simulink model "YMBOX_Control_Core"  (R2024b)
settings: Solver=FixedStepDiscrete  StartTime=0.0  StopTime=3  RelTol=1e-3
PreLoadFcn:
  | run(fullfile(fileparts(get_param(bdroot,'FileName')), 'YMBOX_Deluxe_init.m'));
InitFcn:
  | YMBOX_InitializeModel('core',bdroot);
model workspace (MAT data in the model file):
  KuMDAS_ObserverBuildVariant : Simulink.Parameter (value not decoded)
undefined symbols (not defined in the file or in its folder): CeMDSM_DrvModeIfStart_enum, CeMDSM_DrvModeSpdSens_enum, CeMDSM_DrvModeSpdSmo_enum, CeMDSM_DrvModeTrq_enum, Cf_CONTROL_TASK_TIME_S, KbMDAS_SmoDeadTimeCompEnable_flg, KbMDSA_ActiveInverterCompEnable_flg, KbMDSA_UnifiedVoltageLimitEnable_flg, KbMDSP_DCBusVoltReportFilterEnable_flg, KbMDTM_DAxisPriorityInFW_flg, KbMDTM_FieldWeakeningEnable_flg, KbMDTM_FinalIqAntiWindupEnable_flg, KbMDTM_SensorlessFieldWeakeningEnable_flg, KbMDTM_TorquePriorityBelowBase_flg, KbMDTM_UnifiedConstraintEnable_flg, KfMDAS_ControlCountToElecRad_NULL, KfMDAS_IfAccel_rpms, KfMDAS_IfAlignTime_s, KfMDAS_IfBlendTime_s, KfMDAS_IfSwitchSpd_rpm, KfMDAS_NativeCountToMechRad_NULL, KfMDAS_ObserverExitRatio_NULL, KfMDAS_SlsCtrlPeriod_s, KfMDAS_SlsEAngleInit_rad, KfMDAS_SlsElecSpdMax_rads, KfMDAS_SlsElecSpdMin_rads, KfMDAS_SlsTwoPi_rad, KfMDAS_SmoAngleOffset_rad, KfMDAS_SmoCurrentZohCoefA_NULL, KfMDAS_SmoCurrentZohCoefB_AperV, KfMDAS_SmoDeadTimeCurrentBoundary_A, KfMDAS_SmoDeadTimeDuty_NULL, KfMDAS_SmoDeadTimePolarity_NULL, KfMDAS_SmoDeviceDrop_V, KfMDAS_SmoEmfLpfCoefA_NULL, KfMDAS_SmoEmfLpfCoefB_NULL, KfMDAS_SmoEmfLpfInvPole_s, KfMDAS_SmoErrBoundaryMax_A, KfMDAS_SmoErrBoundarySpan_A, KfMDAS_SmoGainSchedAlpha_NULL, KfMDAS_SmoGainSchedAngleComp_rad, KfMDAS_SmoGainSchedEmfLow_V, KfMDAS_SmoGainSchedInvSpan_PerV, KfMDAS_SmoLdMinusLq_H, KfMDAS_SmoPllKiTs_NULL, KfMDAS_SmoPllKp_NULL, KfMDAS_SmoPllMinEmf_V, KfMDAS_SmoPllSpeedLpfAlpha_NULL, KfMDAS_SmoSlideGainMin_V, KfMDAS_SmoSlideGainSpan_V, KfMDAS_SmoSwitchSpd_rpm, KfMDAS_SmoTotalDelay_s, KfMDCC_DqSoftwareOverCurrentThreshold_A, KfMDCC_PiKcTsId_NULL, KfMDCC_PiKcTsIq_NULL, KfMDCC_PiKiTsId_NULL, KfMDCC_PiKiTsIq_NULL, KfMDCC_PiKpValueId_NULL, KfMDCC_PiKpValueIq_NULL, KfMDCC_PwmFreq_Hz ... (+84)
libraries: YMBOX_SharedMath_Lib x11, spsabctoAlphaBetaZeroLib x1
(part 4 of 8)

== system YMBOX_Control_Core/MDSM/MDSM_ModeManager/MDSM_RouteConfig_Variant ==
  note: 1) Add Subsystem or Model blocks as valid variant choices.
      | 2) You cannot connect blocks at this level. At simulation, connectivity is automatically
      | determined, based on the active variant and port name matching.
  VeMDSM_DrvModeReq_enum : Inport
  VbMDAS_SmoReady_flg : Inport  Port=2
  Route_Variant0_SensoredOnly : Subsystem  VariantControl=KuMDAS_ObserverBuildVariant == 0
      settings: AttributesFormatString=PRODUCT VARIANT 0: SENSORED ROUTE
  Route_Variant1_SMO : Subsystem  VariantControl=KuMDAS_ObserverBuildVariant == 1
      settings: AttributesFormatString=PRODUCT VARIANT 1: I/F TO SMO
  VbMDSM_RouteSupported_flg : Outport
  VbMDSM_Stage1Ready_flg : Outport  Port=2
  VbMDSM_Stage2Enable_flg : Outport  Port=3
  VbMDSM_Stage2Fallback_flg : Outport  Port=4
  VbMDSM_Stage2Ready_flg : Outport  Port=5
  VeMDSM_Stage1Mode_enum : Outport  Port=6
  VeMDSM_Stage2Mode_enum : Outport  Port=7
  VfMDSM_Stage1SwitchSpd_rpm : Outport  Port=8
  VfMDSM_Stage2SwitchSpd_rpm : Outport  Port=9
  VuMDSM_Stage1Acquire_cnt : Outport  Port=10

== system YMBOX_Control_Core/MDSM/MDSM_ModeManager/MDSM_Supervisor_Variant ==
  note: 1) Add Subsystem or Model blocks as valid variant choices.
      | 2) You cannot connect blocks at this level. At simulation, connectivity is automatically
      | determined, based on the active variant and port name matching.
  VbMDSM_MCUEnb_flg : Inport
  VbMDSM_RouteSupported_flg : Inport  Port=2
  VbMDSM_Stage1Ready_flg : Inport  Port=3
  VbMDSM_Stage2Enable_flg : Inport  Port=4
  VbMDSM_Stage2Fallback_flg : Inport  Port=5
  VbMDSM_Stage2Ready_flg : Inport  Port=6
  VeMDSM_DrvModeReq_enum : Inport  Port=7
  VeMDSM_Stage1Mode_enum : Inport  Port=8
  VeMDSM_Stage2Mode_enum : Inport  Port=9
  VfMDSM_Stage1SwitchSpd_rpm : Inport  Port=10
  VfMDSM_Stage2SwitchSpd_rpm : Inport  Port=11
  VfMDSM_TrgtSpd_rpm : Inport  Port=12
  VuMDSM_Stage1Acquire_cnt : Inport  Port=13
  MDSM_Supervisor_SMO : Subsystem  VariantControl=KuMDAS_ObserverBuildVariant == 1
      settings: AttributesFormatString=PRODUCT SUPERVISOR\nMODE 6: I/F -> SMO
  MDSM_Supervisor_SensoredOnly : Subsystem  VariantControl=KuMDAS_ObserverBuildVariant == 0
      settings: AttributesFormatString=|
      | SENSORED ONLY
      | OFF + direct runtime modes 1..5
  VbMDCC_PiReset_flg : Outport
  VbMDTM_PiReset_flg : Outport  Port=2
  VeMDSM_DrvModeCmd_enum : Outport  Port=3
  VuMDFM_FFEnable_enum : Outport  Port=4

== system YMBOX_Control_Core/MDSP/DCBus_Current_Source_Variant/EstimatedFromFOC ==
  physicalCurrent_A : Inport  OutDataTypeStr=single
  dutyU_NULL : Inport  Port=2  OutDataTypeStr=single
  dutyV_NULL : Inport  Port=3  OutDataTypeStr=single
  dutyW_NULL : Inport  Port=4  OutDataTypeStr=single
  phaseU_A : Inport  Port=5  OutDataTypeStr=single
  phaseV_A : Inport  Port=6  OutDataTypeStr=single
  phaseW_A : Inport  Port=7  OutDataTypeStr=single
  phaseSampleValid_flg : Inport  Port=8  OutDataTypeStr=boolean
  CurrentPlausibleMax : Constant  Value=KfMDSP_DCBusCurPlausibleMax_A
  DutyTimesPhaseU : Product  Inputs=**
  DutyTimesPhaseV : Product  Inputs=**
  DutyTimesPhaseW : Product  Inputs=**
  EstimateAndSamplesValid : Logic  IconShape=distinctive
  EstimatedCurrentAbs : Abs
  EstimatedCurrentPlausible : RelationalOperator  Operator=<=
  EstimatedDCBusCurrent : Sum  Inputs=+++
  EstimatedSourceEnum : Constant  Value=uint8(1)  OutDataTypeStr=uint8
  Unused_PhysicalCurrent : Terminator
  currentRaw_A : Outport  OutDataTypeStr=single
  currentValid_flg : Outport  Port=2  OutDataTypeStr=boolean
  sourceEnum : Outport  Port=3  OutDataTypeStr=uint8
  wires:
  physicalCurrent_A/1 -> Unused_PhysicalCurrent/1
  EstimatedSourceEnum/1 -> sourceEnum/1
  EstimateAndSamplesValid/1 -> currentValid_flg/1
  phaseSampleValid_flg/1 -> EstimateAndSamplesValid/2
  EstimatedCurrentPlausible/1 -> EstimateAndSamplesValid/1
  CurrentPlausibleMax/1 -> EstimatedCurrentPlausible/2
  EstimatedCurrentAbs/1 -> EstimatedCurrentPlausible/1
  EstimatedDCBusCurrent/1 -> currentRaw_A/1, EstimatedCurrentAbs/1
  DutyTimesPhaseW/1 -> EstimatedDCBusCurrent/3
  DutyTimesPhaseV/1 -> EstimatedDCBusCurrent/2
  DutyTimesPhaseU/1 -> EstimatedDCBusCurrent/1
  phaseW_A/1 -> DutyTimesPhaseW/2
  dutyW_NULL/1 -> DutyTimesPhaseW/1
  phaseV_A/1 -> DutyTimesPhaseV/2
  dutyV_NULL/1 -> DutyTimesPhaseV/1
  phaseU_A/1 -> DutyTimesPhaseU/2
  dutyU_NULL/1 -> DutyTimesPhaseU/1

== system YMBOX_Control_Core/MDSP/DCBus_Current_Source_Variant/PhysicalSensor ==
  physicalCurrent_A : Inport  OutDataTypeStr=single
  dutyU_NULL : Inport  Port=2  OutDataTypeStr=single
  dutyV_NULL : Inport  Port=3  OutDataTypeStr=single
  dutyW_NULL : Inport  Port=4  OutDataTypeStr=single
  phaseU_A : Inport  Port=5  OutDataTypeStr=single
  phaseV_A : Inport  Port=6  OutDataTypeStr=single
  phaseW_A : Inport  Port=7  OutDataTypeStr=single
  phaseSampleValid_flg : Inport  Port=8  OutDataTypeStr=boolean
  CurrentPlausibleMax : Constant  Value=KfMDSP_DCBusCurPlausibleMax_A
  PhysicalCurrentAbs : Abs
  PhysicalCurrentPlausible : RelationalOperator  Operator=<=
  PhysicalSourceEnum : Constant  Value=uint8(0)  OutDataTypeStr=uint8
  Unused_DutyU : Terminator
  Unused_DutyV : Terminator
  Unused_DutyW : Terminator
  Unused_PhaseU : Terminator
  Unused_PhaseV : Terminator
  Unused_PhaseValid : Terminator
  Unused_PhaseW : Terminator
  currentRaw_A : Outport  OutDataTypeStr=single
  currentValid_flg : Outport  Port=2  OutDataTypeStr=boolean
  sourceEnum : Outport  Port=3  OutDataTypeStr=uint8
  wires:
  phaseSampleValid_flg/1 -> Unused_PhaseValid/1
  phaseW_A/1 -> Unused_PhaseW/1
  phaseV_A/1 -> Unused_PhaseV/1
  phaseU_A/1 -> Unused_PhaseU/1
  dutyW_NULL/1 -> Unused_DutyW/1
  dutyV_NULL/1 -> Unused_DutyV/1
  dutyU_NULL/1 -> Unused_DutyU/1
  PhysicalSourceEnum/1 -> sourceEnum/1
  PhysicalCurrentPlausible/1 -> currentValid_flg/1
  CurrentPlausibleMax/1 -> PhysicalCurrentPlausible/2
  PhysicalCurrentAbs/1 -> PhysicalCurrentPlausible/1
  physicalCurrent_A/1 -> currentRaw_A/1, PhysicalCurrentAbs/1

== system YMBOX_Control_Core/MDTM/Command_Constraint_FieldWeakening_Manager/Command_Diagnostics ==
  iqCmd : Inport
  idCmd : Inport  Port=2
  currentMax : Inport  Port=3
  omegaElec : Inport  Port=4
  vmax : Inport  Port=5
  rs : Inport  Port=6
  ld : Inport  Port=7
  lq : Inport  Port=8
  pmFlux : Inport  Port=9
  polePairs : Inport  Port=10
  modeCmd : Inport  Port=11
  Calculate_Command_Diagnostics : MATLAB Function  Description=Calculate final current/voltage utilization, torque estimate, and equivalent-Iq anti-windup feedback.  TreatAsAtomicUnit=on
  currentUtilization : Outport
  voltageUtilization : Outport  Port=2
  iqAntiWindupFeedback : Outport  Port=3
  torqueEstimate_Nm : Outport  Port=4
  wires:
  vmax/1 -> Calculate_Command_Diagnostics/5(vmax)
  iqCmd/1 -> Calculate_Command_Diagnostics/1(iqCmd)
  rs/1 -> Calculate_Command_Diagnostics/6(rs)
  idCmd/1 -> Calculate_Command_Diagnostics/2(idCmd)
  ld/1 -> Calculate_Command_Diagnostics/7(ld)
  currentMax/1 -> Calculate_Command_Diagnostics/3(currentMax)
  lq/1 -> Calculate_Command_Diagnostics/8(lq)
  omegaElec/1 -> Calculate_Command_Diagnostics/4(omegaElec)
  pmFlux/1 -> Calculate_Command_Diagnostics/9(pmFlux)
  polePairs/1 -> Calculate_Command_Diagnostics/10(polePairs)
  modeCmd/1 -> Calculate_Command_Diagnostics/11(modeCmd)
  Calculate_Command_Diagnostics/1(currentUtilization) -> currentUtilization/1  "currentUtilization"
  Calculate_Command_Diagnostics/2(voltageUtilization) -> voltageUtilization/1  "voltageUtilization"
  Calculate_Command_Diagnostics/3(iqAntiWindupFeedback) -> iqAntiWindupFeedback/1  "iqAntiWindupFeedback"
  Calculate_Command_Diagnostics/4(torqueEstimate_Nm) -> torqueEstimate_Nm/1  "torqueEstimate_Nm"

== system YMBOX_Control_Core/MDTM/Command_Constraint_FieldWeakening_Manager/Current_Vector_Constraint ==
  iqRaw : Inport
  idRaw : Inport  Port=2
  idRequest : Inport  Port=3
  fwActive : Inport  Port=4
  unifiedEnable : Inport  Port=5
  currentMax : Inport  Port=6
  torquePriority : Inport  Port=7
  dAxisPriority : Inport  Port=8
  modeCmd : Inport  Port=9
  Apply_Current_Vector_Constraint : MATLAB Function  Description=Apply unified current-circle constraint with torque priority below base speed and d-axis priority during field weakening.  TreatAsAtomicUnit=on
  iqCmd : Outport
  idCmd : Outport  Port=2
  iqLimit : Outport  Port=3
  currentLimited : Outport  Port=4
  wires:
  unifiedEnable/1 -> Apply_Current_Vector_Constraint/5(unifiedEnable)
  iqRaw/1 -> Apply_Current_Vector_Constraint/1(iqRaw)
  currentMax/1 -> Apply_Current_Vector_Constraint/6(currentMax)
  idRaw/1 -> Apply_Current_Vector_Constraint/2(idRaw)
  torquePriority/1 -> Apply_Current_Vector_Constraint/7(torquePriority)
  idRequest/1 -> Apply_Current_Vector_Constraint/3(idRequest)
  dAxisPriority/1 -> Apply_Current_Vector_Constraint/8(dAxisPriority)
  fwActive/1 -> Apply_Current_Vector_Constraint/4(fwActive)
  modeCmd/1 -> Apply_Current_Vector_Constraint/9(modeCmd)
  Apply_Current_Vector_Constraint/1(iqCmd) -> iqCmd/1  "iqCmd"
  Apply_Current_Vector_Constraint/2(idCmd) -> idCmd/1  "idCmd"
  Apply_Current_Vector_Constraint/3(iqLimit) -> iqLimit/1  "iqLimit"
  Apply_Current_Vector_Constraint/4(currentLimited) -> currentLimited/1  "currentLimited"

== system YMBOX_Control_Core/MDTM/Command_Constraint_FieldWeakening_Manager/Field_Weakening_Controller ==
  idRaw : Inport
  iqRaw : Inport  Port=2
  rpmAbs : Inport  Port=3
  omegaElec : Inport  Port=4
  vmax : Inport  Port=5
  utilRaw : Inport  Port=6
  fwAllowed : Inport  Port=7  OutDataTypeStr=boolean
  modeCmd : Inport  Port=8
  ld : Inport  Port=9
  lq : Inport  Port=10
  pmFlux : Inport  Port=11
  fwEntryUtil : Inport  Port=12
  fwExitUtil : Inport  Port=13
  fwEntrySpeedRpm : Inport  Port=14
  fwIdMin : Inport  Port=15
  fwKp : Inport  Port=16
  fwKiTs : Inport  Port=17
  fwIdSlew : Inport  Port=18
  FW_Id_Memory : UnitDelay  Description=Previous slew-limited field-weakening Id contribution.  InitialCondition=single(0)  SampleTime=-1
  FW_Integrator_Memory : UnitDelay  Description=Previous weak-field voltage-loop integrator.  InitialCondition=single(0)  SampleTime=-1
  FW_State_Memory : UnitDelay  Description=Previous field-weakening latch state.  InitialCondition=false  SampleTime=-1
  Field_Weakening_State_Update : MATLAB Function  Description=Pure next-state and output calculation. State storage remains visible in Unit Delay blocks.  TreatAsAtomicUnit=on
  idRequest : Outport
  fwActive : Outport  Port=2
  fwIdContribution : Outport  Port=3
  wires:
  vmax/1 -> Field_Weakening_State_Update/5(vmax)
  idRaw/1 -> Field_Weakening_State_Update/1(idRaw)
  utilRaw/1 -> Field_Weakening_State_Update/6(utilRaw)
  Field_Weakening_State_Update/6(fwIdContribution) -> fwIdContribution/1  "fwIdContribution"
  iqRaw/1 -> Field_Weakening_State_Update/2(iqRaw)
  fwAllowed/1 -> Field_Weakening_State_Update/7(fwAllowed)
  rpmAbs/1 -> Field_Weakening_State_Update/3(rpmAbs)
  modeCmd/1 -> Field_Weakening_State_Update/8(modeCmd)
  FW_State_Memory/1 -> Field_Weakening_State_Update/19(fwStatePrev)  "fwStatePrev"
  omegaElec/1 -> Field_Weakening_State_Update/4(omegaElec)
  ld/1 -> Field_Weakening_State_Update/9(ld)
  lq/1 -> Field_Weakening_State_Update/10(lq)
  pmFlux/1 -> Field_Weakening_State_Update/11(pmFlux)
  fwEntryUtil/1 -> Field_Weakening_State_Update/12(fwEntryUtil)
  fwExitUtil/1 -> Field_Weakening_State_Update/13(fwExitUtil)
  fwEntrySpeedRpm/1 -> Field_Weakening_State_Update/14(fwEntrySpeedRpm)
  Field_Weakening_State_Update/4(idRequest) -> idRequest/1  "idRequest"
  fwIdMin/1 -> Field_Weakening_State_Update/15(fwIdMin)
  fwKp/1 -> Field_Weakening_State_Update/16(fwKp)
  fwKiTs/1 -> Field_Weakening_State_Update/17(fwKiTs)
  fwIdSlew/1 -> Field_Weakening_State_Update/18(fwIdSlew)
  Field_Weakening_State_Update/1(fwStateNext) -> FW_State_Memory/1  "fwStateNext"
  Field_Weakening_State_Update/2(fwIntegratorNext) -> FW_Integrator_Memory/1  "fwIntegratorNext"
  Field_Weakening_State_Update/3(fwIdStateNext) -> FW_Id_Memory/1  "fwIdStateNext"
  Field_Weakening_State_Update/5(fwActive) -> fwActive/1  "fwActive"
  FW_Integrator_Memory/1 -> Field_Weakening_State_Update/20(fwIntegratorPrev)  "fwIntegratorPrev"
  FW_Id_Memory/1 -> Field_Weakening_State_Update/21(fwIdStatePrev)  "fwIdStatePrev"

== system YMBOX_Control_Core/MDTM/Command_Constraint_FieldWeakening_Manager/Field_Weakening_Permission ==
  modeCmd : Inport
  reset : Inport  Port=2  OutDataTypeStr=boolean
  vdc : Inport  Port=3
  minValidVdc : Inport  Port=4
  fwSensoredEnable : Inport  Port=5  OutDataTypeStr=boolean
  fwSensorlessEnable : Inport  Port=6  OutDataTypeStr=boolean
  speedValid : Inport  Port=7  OutDataTypeStr=boolean
  positionQuality : Inport  Port=8
  minPositionQuality : Inport  Port=9
  Allowed : Logic  Inputs=5  IconShape=distinctive
  LowVoltage : RelationalOperator  Operator=<
  MaxMode : RelationalOperator  Operator=<=
  MinMode : RelationalOperator
  ModeMax : Constant  Value=5  OutDataTypeStr=uint16
  ModeMin : Constant  OutDataTypeStr=uint16
  ModeOk : Logic  Operator=OR  IconShape=distinctive
  NoReset : Logic  Operator=NOT  Inputs=1  IconShape=distinctive
  Quality : RelationalOperator
  Sensored : Logic  Inputs=3  IconShape=distinctive
  Sensorless : Logic  IconShape=distinctive
  SensorlessMin : Constant  Value=16  OutDataTypeStr=uint16
  SlMode : RelationalOperator
  VoltageOk : Logic  Operator=NOT  Inputs=1  IconShape=distinctive
  fwAllowed : Outport  OutDataTypeStr=boolean
  wires:
  MaxMode/1 -> Sensored/2
  ModeMin/1 -> MinMode/2
  fwSensoredEnable/1 -> Sensored/3
  modeCmd/1 -> MaxMode/1, MinMode/1, SlMode/1
  SensorlessMin/1 -> SlMode/2
  ModeMax/1 -> MaxMode/2
  MinMode/1 -> Sensored/1
  SlMode/1 -> Sensorless/1
  fwSensorlessEnable/1 -> Sensorless/2
  vdc/1 -> LowVoltage/1
  minValidVdc/1 -> LowVoltage/2
  Sensored/1 -> ModeOk/1
  Sensorless/1 -> ModeOk/2
  reset/1 -> NoReset/1
  LowVoltage/1 -> VoltageOk/1
  positionQuality/1 -> Quality/1
  minPositionQuality/1 -> Quality/2
  ModeOk/1 -> Allowed/1
  NoReset/1 -> Allowed/2
  VoltageOk/1 -> Allowed/3
  speedValid/1 -> Allowed/4
  Quality/1 -> Allowed/5
  Allowed/1 -> fwAllowed/1

== system YMBOX_Control_Core/MDTM/Command_Constraint_FieldWeakening_Manager/Operating_Point_Estimator ==
  iqRaw : Inport
  idRaw : Inport  Port=2
  speedRads : Inport  Port=3
  vdc : Inport  Port=4
  vdqMaxPerVdc : Inport  Port=5
  rs : Inport  Port=6
  ld : Inport  Port=7
  lq : Inport  Port=8
  pmFlux : Inport  Port=9
  polePairs : Inport  Port=10
  modeCmd : Inport  Port=11
  fwAllowed : Inport  Port=12  OutDataTypeStr=boolean
  Estimate_Operating_Point : MATLAB Function  Description=Estimate mechanical speed, electrical speed, available dq voltage, and pre-constraint voltage utilization.  TreatAsAtomicUnit=on
  rpmAbs : Outport
  omegaElec : Outport  Port=2
  vmax : Outport  Port=3
  utilRaw : Outport  Port=4
  wires:
  vdqMaxPerVdc/1 -> Estimate_Operating_Point/5(vdqMaxPerVdc)
  iqRaw/1 -> Estimate_Operating_Point/1(iqRaw)
  rs/1 -> Estimate_Operating_Point/6(rs)
  idRaw/1 -> Estimate_Operating_Point/2(idRaw)
  ld/1 -> Estimate_Operating_Point/7(ld)
  speedRads/1 -> Estimate_Operating_Point/3(speedRads)
  lq/1 -> Estimate_Operating_Point/8(lq)
  vdc/1 -> Estimate_Operating_Point/4(vdc)
  pmFlux/1 -> Estimate_Operating_Point/9(pmFlux)
  polePairs/1 -> Estimate_Operating_Point/10(polePairs)
  modeCmd/1 -> Estimate_Operating_Point/11(modeCmd)
  fwAllowed/1 -> Estimate_Operating_Point/12(fwAllowed)
  Estimate_Operating_Point/4(utilRaw) -> utilRaw/1  "utilRaw"
  Estimate_Operating_Point/1(rpmAbs) -> rpmAbs/1  "rpmAbs"
  Estimate_Operating_Point/2(omegaElec) -> omegaElec/1  "omegaElec"
  Estimate_Operating_Point/3(vmax) -> vmax/1  "vmax"

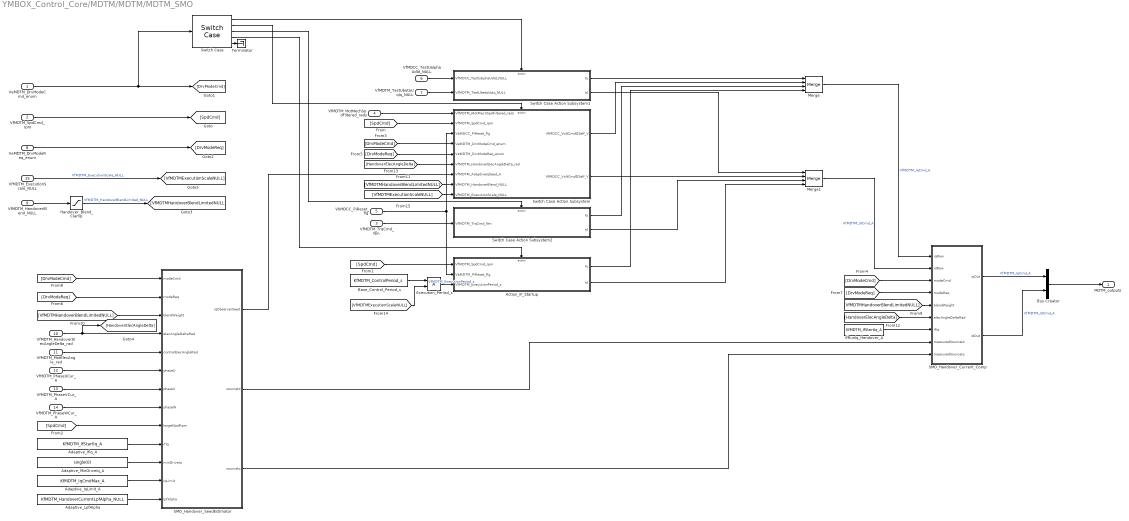
== system YMBOX_Control_Core/MDTM/MDTM/MDTM_SMO ==
  VeMDTM_DrvModeCmd_enum : Inport
  VfMDTM_SpdCmd_rpm : Inport  Port=2
  VfMDTM_TrqCmd_Nm : Inport  Port=3
  VfMDTM_MotMechSpdFiltered_rads : Inport  Port=4
  VbMDCC_PiReset_flg : Inport  Port=5
  VfMDCC_TestUalphaUdId_NULL : Inport  Port=6
  VfMDTM_TestUbetaUqIq_NULL : Inport  Port=7
  VeMDTM_DrvModeReq_enum : Inport  Port=8
  VfMDTM_HandoverBlend_NULL : Inport  Port=9
  VfMDTM_HandoverElecAngleDelta_rad : Inport  Port=10
  VfMDTM_MotElecAngle_rad : Inport  Port=11
  VfMDTM_PhaseUCur_A : Inport  Port=12
  VfMDTM_PhaseVCur_A : Inport  Port=13
  VfMDTM_PhaseWCur_A : Inport  Port=14
  VfMDTM_ExecutionScale_NULL : Inport  Port=15  OutDataTypeStr=single
  Action_IF_Startup : Subsystem  TreatAsAtomicUnit=on
  Adaptive_IfIq_A : Constant  Value=KfMDTM_IfStartIq_A
  Adaptive_IqLimit_A : Constant  Value=KfMDTM_IqCmdMax_A
  Adaptive_LpfAlpha : Constant  Value=KfMDTM_HandoverCurrentLpfAlpha_NULL
  Adaptive_MinDriveIq_A : Constant  Description=Handover must preserve the measured torque current. A fixed acceleration-current floor injects torque under a light load.  Value=single(0)
  Base_Control_Period_s : Constant  Value=KfMDTM_ControlPeriod_s  OutDataTypeStr=single
  Bus Creator : BusCreator  Inputs=2
  Execution_Period_s : Product  Inputs=**
  Handover_Blend_Clamp : Saturate  UpperLimit=single(1)  LowerLimit=single(0)  OutDataTypeStr=single
  IfRunIq_Handover_A : Constant  Value=KfMDTM_IfStartIq_A
  Merge : Merge  Inputs=4
  Merge1 : Merge  Inputs=4
  SMO_Handover_Current_Comp : Subsystem
  SMO_Handover_SeedEstimator : Subsystem
  Switch Case : SwitchCase  CaseConditions={CeMDSM_DrvModeCurrDQ_enum,[CeMDSM_DrvModeSpdSens_enum,CeMDSM_DrvModeSpdSmo_enum],CeMDSM_DrvModeTrq_enum,CeMDSM_DrvModeIfStart_enum}
      settings: AttributesFormatString=PRODUCT MODES\n3 TEST | 4/17 SPEED | 5 TORQUE | 16 I/F
  Switch Case Action Subsystem : Subsystem  TreatAsAtomicUnit=on
  Switch Case Action Subsystem1 : Subsystem  TreatAsAtomicUnit=on
  Switch Case Action Subsystem2 : Subsystem  TreatAsAtomicUnit=on
  Terminator : Terminator
  MDTM_outputs : Outport
  wires:
  Merge/1 -> SMO_Handover_Current_Comp/1(iqRaw)  "VfMDTM_IqCmd_A"
  VfMDTM_HandoverBlend_NULL/1 -> Handover_Blend_Clamp/1
  Adaptive_IqLimit_A/1 -> SMO_Handover_SeedEstimator/12(iqLimit)
  VeMDTM_DrvModeCmd_enum/1 -> Switch Case/1, [DrvModeCmd]
  SMO_Handover_SeedEstimator/3(sourceIq) -> SMO_Handover_Current_Comp/9(measuredSourceIq)
  VfMDTM_HandoverElecAngleDelta_rad/1 -> [HandoverElecAngleDelta], SMO_Handover_SeedEstimator/4(elecAngleDeltaRad)
  Adaptive_LpfAlpha/1 -> SMO_Handover_SeedEstimator/13(lpfAlpha)
  VfMDTM_MotElecAngle_rad/1 -> SMO_Handover_SeedEstimator/5(controlElecAngleRad)
  Merge1/1 -> SMO_Handover_Current_Comp/2(idRaw)  "VfMDTM_IdCmd_A"
  VfMDTM_PhaseUCur_A/1 -> SMO_Handover_SeedEstimator/6(phaseU)
  VfMDTM_PhaseVCur_A/1 -> SMO_Handover_SeedEstimator/7(phaseV)
  VfMDTM_PhaseWCur_A/1 -> SMO_Handover_SeedEstimator/8(phaseW)
  Adaptive_IfIq_A/1 -> SMO_Handover_SeedEstimator/10(ifIq)
  VfMDTM_TrqCmd_Nm/1 -> Switch Case Action Subsystem2/1(VfMDTM_TrqCmd_Nm)
  Adaptive_MinDriveIq_A/1 -> SMO_Handover_SeedEstimator/11(minDriveIq)
  Bus Creator/1 -> MDTM_outputs/1
  VfMDCC_TestUalphaUdId_NULL/1 -> Switch Case Action Subsystem1/1(VfMDCC_TestUalphaUdId_NULL)
  SMO_Handover_Current_Comp/2(idOut) -> Bus Creator/2  "VfMDTM_IdCmd_A"
  IfRunIq_Handover_A/1 -> SMO_Handover_Current_Comp/7(ifIq)
  VfMDTM_TestUbetaUqIq_NULL/1 -> Switch Case Action Subsystem1/2(VfMDTM_TestUbetaUqIq_NULL)
  VfMDTM_MotMechSpdFiltered_rads/1 -> Switch Case Action Subsystem/1(VfMDTM_MotMechSpdFiltered_rads)
  Switch Case/1 -> Switch Case Action Subsystem1/Action
  Switch Case/3 -> Switch Case Action Subsystem2/Action
  Switch Case/2 -> Switch Case Action Subsystem/Action
  Switch Case/5 -> Terminator/1
  Switch Case/4 -> Action_IF_Startup/Action
  VbMDCC_PiReset_flg/1 -> Action_IF_Startup/2(VbMDTM_PiReset_flg), Switch Case Action Subsystem/3(VbMDCC_PiReset_flg)
  SMO_Handover_SeedEstimator/1(iqObserverSeed) -> Switch Case Action Subsystem/7(VfMDTM_AdaptiveIqSeed_A)
  SMO_Handover_SeedEstimator/2(sourceId) -> SMO_Handover_Current_Comp/8(measuredSourceId)
  Switch Case Action Subsystem1/2(Id) -> Merge1/1
  Switch Case Action Subsystem1/1(Iq) -> Merge/1
  Switch Case Action Subsystem/2(VfMDCC_VoltCmdDSelf_V) -> Merge1/2
  Switch Case Action Subsystem/1(VfMDCC_VoltCmdQSelf_V) -> Merge/2
  Switch Case Action Subsystem2/2(Id) -> Merge1/3
  Switch Case Action Subsystem2/1(Iq) -> Merge/3
  Action_IF_Startup/2(Id) -> Merge1/4
  Action_IF_Startup/1(Iq) -> Merge/4
  SMO_Handover_Current_Comp/1(iqOut) -> Bus Creator/1  "VfMDTM_IqCmd_A"
  VfMDTM_SpdCmd_rpm/1 -> [SpdCmd]
  [SpdCmd] -> Switch Case Action Subsystem/2(VfMDTM_SpdCmd_rpm)
  [SpdCmd] -> Action_IF_Startup/1(VfMDTM_SpdCmd_rpm)
  [SpdCmd] -> SMO_Handover_SeedEstimator/9(targetSpdRpm)
  [DrvModeCmd] -> Switch Case Action Subsystem/4(VeMDTM_DrvModeCmd_enum)
  [DrvModeCmd] -> SMO_Handover_Current_Comp/3(modeCmd)
  VeMDTM_DrvModeReq_enum/1 -> [DrvModeReq]
  [DrvModeReq] -> Switch Case Action Subsystem/5(VeMDTM_DrvModeReq_enum)
  [DrvModeReq] -> SMO_Handover_SeedEstimator/2(modeReq)
  [DrvModeReq] -> SMO_Handover_Current_Comp/4(modeReq)
  [DrvModeCmd] -> SMO_Handover_SeedEstimator/1(modeCmd)
  Base_Control_Period_s/1 -> Execution_Period_s/1
  Execution_Period_s/1 -> Action_IF_Startup/3(VfMDTM_ExecutionPeriod_s)  "VfMDTM_ExecutionPeriod_s"
  Handover_Blend_Clamp/1 -> [VfMDTMHandoverBlendLimitedNULL]  "VfMDTM_HandoverBlendLimited_NULL"
  [VfMDTMHandoverBlendLimitedNULL] -> SMO_Handover_Current_Comp/5(blendWeight)
  [VfMDTMHandoverBlendLimitedNULL] -> SMO_Handover_SeedEstimator/3(blendWeight)
  [VfMDTMHandoverBlendLimitedNULL] -> Switch Case Action Subsystem/8(VfMDTM_HandoverBlend_NULL)
  [HandoverElecAngleDelta] -> SMO_Handover_Current_Comp/6(elecAngleDeltaRad)
  [HandoverElecAngleDelta] -> Switch Case Action Subsystem/6(VfMDTM_HandoverElecAngleDelta_rad)
  VfMDTM_ExecutionScale_NULL/1 -> [VfMDTMExecutionScaleNULL]  "VfMDTM_ExecutionScale_NULL"
  [VfMDTMExecutionScaleNULL] -> Execution_Period_s/2
  [VfMDTMExecutionScaleNULL] -> Switch Case Action Subsystem/9(VfMDTM_ExecutionScale_NULL)

== system YMBOX_Control_Core/MDTM/MDTM/MDTM_SensoredOnly ==
  VeMDTM_DrvModeCmd_enum : Inport
  VfMDTM_SpdCmd_rpm : Inport  Port=2
  VfMDTM_TrqCmd_Nm : Inport  Port=3
  VfMDTM_MotMechSpdFiltered_rads : Inport  Port=4
  VbMDCC_PiReset_flg : Inport  Port=5
  VfMDCC_TestUalphaUdId_NULL : Inport  Port=6
  VfMDTM_TestUbetaUqIq_NULL : Inport  Port=7
  VeMDTM_DrvModeReq_enum : Inport  Port=8
  VfMDTM_HandoverBlend_NULL : Inport  Port=9
  VfMDTM_HandoverElecAngleDelta_rad : Inport  Port=10
  VfMDTM_MotElecAngle_rad : Inport  Port=11
  VfMDTM_PhaseUCur_A : Inport  Port=12
  VfMDTM_PhaseVCur_A : Inport  Port=13
  VfMDTM_PhaseWCur_A : Inport  Port=14
  VfMDTM_ExecutionScale_NULL : Inport  Port=15  OutDataTypeStr=single
  Bus Creator : BusCreator  Inputs=2
  Merge : Merge  Inputs=3
  Merge1 : Merge  Inputs=3
  Switch Case : SwitchCase  CaseConditions={CeMDSM_DrvModeCurrDQ_enum,CeMDSM_DrvModeSpdSens_enum,CeMDSM_DrvModeTrq_enum}
  Switch Case Action Subsystem : Subsystem  TreatAsAtomicUnit=on
      settings: AttributesFormatString=|
      | SENSORED SPEED PI
      | Measured-speed command-ramp seed; zero PI reset seed
  Switch Case Action Subsystem1 : Subsystem  TreatAsAtomicUnit=on
  Switch Case Action Subsystem2 : Subsystem  TreatAsAtomicUnit=on
  TerminateInput08 : Terminator
  TerminateInput09 : Terminator
  TerminateInput{10..14} (5 alike) : Terminator
  Terminator : Terminator
  MDTM_outputs : Outport
  wires:
  VeMDTM_DrvModeCmd_enum/1 -> Switch Case/1
  Switch Case/1 -> Switch Case Action Subsystem1/Action
  Switch Case/2 -> Switch Case Action Subsystem/Action
  Switch Case/3 -> Switch Case Action Subsystem2/Action
  Switch Case/4 -> Terminator/1
  VfMDCC_TestUalphaUdId_NULL/1 -> Switch Case Action Subsystem1/1(VfMDCC_TestUalphaUdId_NULL)
  VfMDTM_TestUbetaUqIq_NULL/1 -> Switch Case Action Subsystem1/2(VfMDTM_TestUbetaUqIq_NULL)
  VfMDTM_MotMechSpdFiltered_rads/1 -> Switch Case Action Subsystem/1(VfMDTM_MotMechSpdFiltered_rads)
  VfMDTM_SpdCmd_rpm/1 -> Switch Case Action Subsystem/2(VfMDTM_SpdCmd_rpm)
  VbMDCC_PiReset_flg/1 -> Switch Case Action Subsystem/3(VbMDCC_PiReset_flg)
  VfMDTM_TrqCmd_Nm/1 -> Switch Case Action Subsystem2/1(VfMDTM_TrqCmd_Nm)
  Switch Case Action Subsystem1/1(Iq) -> Merge/1
  Switch Case Action Subsystem/1(VfMDCC_VoltCmdQSelf_V) -> Merge/2
  Switch Case Action Subsystem2/1(Iq) -> Merge/3
  Switch Case Action Subsystem1/2(Id) -> Merge1/1
  Switch Case Action Subsystem/2(VfMDCC_VoltCmdDSelf_V) -> Merge1/2
  Switch Case Action Subsystem2/2(Id) -> Merge1/3
  Merge/1 -> Bus Creator/1  "VfMDTM_IqCmd_A"
  Merge1/1 -> Bus Creator/2  "VfMDTM_IdCmd_A"
  Bus Creator/1 -> MDTM_outputs/1
  VeMDTM_DrvModeReq_enum/1 -> TerminateInput08/1
  VfMDTM_HandoverBlend_NULL/1 -> TerminateInput09/1
  VfMDTM_HandoverElecAngleDelta_rad/1 -> TerminateInput10/1
  VfMDTM_MotElecAngle_rad/1 -> TerminateInput11/1
  VfMDTM_PhaseUCur_A/1 -> TerminateInput12/1
  VfMDTM_PhaseVCur_A/1 -> TerminateInput13/1
  VfMDTM_PhaseWCur_A/1 -> TerminateInput14/1
  VfMDTM_ExecutionScale_NULL/1 -> Switch Case Action Subsystem/4(VfMDTM_ExecutionScale_NULL)  "VfMDTM_ExecutionScale_NULL"

== system YMBOX_Control_Core/MDTM/MotorCurrentReferenceGenerator/MotorCurrentReference_IPMSM ==
  iqLegacy_A : Inport
  idLegacy_A : Inport  Port=2
  modeCmd_enum : Inport  Port=3
  handoverBlend_NULL : Inport  Port=4  OutDataTypeStr=single
  Abs_EquivalentIq : Abs
  Apply_Torque_Direction : Product  Inputs=**
  EquivalentIq_To_Torque : Gain  Gain=KfMDTM_TorqueConstant_NmPerA  OutDataTypeStr=single
  Handover_Complete : Constant  Value=single(1)  OutDataTypeStr=single
  Is_Handover_Complete : RelationalOperator
  Is_Mode17 : RelationalOperator  Operator===  OutDataTypeStr=boolean
  Is_Mode4 : RelationalOperator  Operator===  OutDataTypeStr=boolean
  Is_Mode5 : RelationalOperator  Operator===  OutDataTypeStr=boolean
  MTPA_Id_Lookup : Lookup_n-D  NumberOfTableDimensions=1  BreakpointsForDimension1=KfMDTM_MTPAEquivalentIqBreakpoints_A  Table=KfMDTM_MTPAIdTable_A  ExtrapMethod=Clip
  MTPA_Iq_Lookup : Lookup_n-D  NumberOfTableDimensions=1  BreakpointsForDimension1=KfMDTM_MTPAEquivalentIqBreakpoints_A  Table=KfMDTM_MTPAIqTable_A  ExtrapMethod=Clip
  MTPA_Mode_Enable : Logic  Operator=OR  Inputs=3  IconShape=distinctive  OutDataTypeStr=boolean
  Mode17_After_Handover : Logic
  Select_Id_Reference : Switch  Criteria=u2 ~= 0
  Select_Iq_Reference : Switch  Criteria=u2 ~= 0
  SensoredSpeedMode : Constant  Value=CeMDSM_DrvModeSpdSens_enum  OutDataTypeStr=uint16
  SmoClosedLoopMode : Constant  Value=CeMDSM_DrvModeSpdSmo_enum  OutDataTypeStr=uint16
  TorqueMode : Constant  Value=CeMDSM_DrvModeTrq_enum  OutDataTypeStr=uint16
  Torque_Direction : Signum
  iqReference_A : Outport
  idReference_A : Outport  Port=2
  torqueRequest_Nm : Outport  Port=3
  mtpaActive_flg : Outport  Port=4
  wires:
  Is_Mode4/1 -> MTPA_Mode_Enable/1
  SensoredSpeedMode/1 -> Is_Mode4/2
  modeCmd_enum/1 -> Is_Mode5/1, Is_Mode17/1, Is_Mode4/1
  Handover_Complete/1 -> Is_Handover_Complete/2
  TorqueMode/1 -> Is_Mode5/2
  iqLegacy_A/1 -> Abs_EquivalentIq/1, EquivalentIq_To_Torque/1, Torque_Direction/1, Select_Iq_Reference/3
  SmoClosedLoopMode/1 -> Is_Mode17/2
  handoverBlend_NULL/1 -> Is_Handover_Complete/1
  Is_Mode5/1 -> MTPA_Mode_Enable/2
  Abs_EquivalentIq/1 -> MTPA_Id_Lookup/1, MTPA_Iq_Lookup/1
  Is_Mode17/1 -> Mode17_After_Handover/1
  Is_Handover_Complete/1 -> Mode17_After_Handover/2
  EquivalentIq_To_Torque/1 -> torqueRequest_Nm/1  "VfMDTM_TorqueRequest_Nm"
  Mode17_After_Handover/1 -> MTPA_Mode_Enable/3
  MTPA_Iq_Lookup/1 -> Apply_Torque_Direction/1
  Torque_Direction/1 -> Apply_Torque_Direction/2
  MTPA_Id_Lookup/1 -> Select_Id_Reference/1
  idLegacy_A/1 -> Select_Id_Reference/3
  MTPA_Mode_Enable/1 -> Select_Id_Reference/2, mtpaActive_flg/1, Select_Iq_Reference/2  "VbMDTM_MtpaActive_flg"
  Apply_Torque_Direction/1 -> Select_Iq_Reference/1
  Select_Id_Reference/1 -> idReference_A/1  "VfMDTM_IdReference_A"
  Select_Iq_Reference/1 -> iqReference_A/1  "VfMDTM_IqReference_A"

== system YMBOX_Control_Core/MDTM/MotorCurrentReferenceGenerator/MotorCurrentReference_SPMSM ==
  iqLegacy_A : Inport
  idLegacy_A : Inport  Port=2
  modeCmd_enum : Inport  Port=3
  handoverBlend_NULL : Inport  Port=4  OutDataTypeStr=single
  EquivalentIq_To_Torque : Gain  Gain=KfMDTM_TorqueConstant_NmPerA  OutDataTypeStr=single
  MTPA_Inactive : Constant  Value=false  OutDataTypeStr=boolean
  Unused_Handover_Blend : Terminator
  Unused_Mode : Terminator
  iqReference_A : Outport
  idReference_A : Outport  Port=2
  torqueRequest_Nm : Outport  Port=3
  mtpaActive_flg : Outport  Port=4
  wires:
  idLegacy_A/1 -> idReference_A/1  "VfMDTM_IdReference_A"
  iqLegacy_A/1 -> iqReference_A/1, EquivalentIq_To_Torque/1  "VfMDTM_IqReference_A"
  MTPA_Inactive/1 -> mtpaActive_flg/1  "VbMDTM_MtpaActive_flg"
  handoverBlend_NULL/1 -> Unused_Handover_Blend/1
  modeCmd_enum/1 -> Unused_Mode/1
  EquivalentIq_To_Torque/1 -> torqueRequest_Nm/1  "VfMDTM_TorqueRequest_Nm"

== system YMBOX_Control_Core/MDAS/MDAS_DriveModeRoute_Variant/MDAS_Route_SMO/Action_DefaultZero ==
  note: delta_cpr_err
  Action Port : ActionPort  ActionPortLabel=default:
  Zero1 : Constant  Value=single(0)  OutDataTypeStr=single
  Zero2 : Constant  Value=single(0)  OutDataTypeStr=single
  Zero3 : Constant  Value=single(0)  OutDataTypeStr=single
  VfMDAS_MotMechSpdFiltered_rads : Outport
  VfMDAS_MotMechSpdFilteredAbs_rads : Outport  Port=2
  VfMDAS_SelectedElecAngle_rad : Outport  Port=3
  wires:
  Zero1/1 -> VfMDAS_MotMechSpdFiltered_rads/1
  Zero2/1 -> VfMDAS_MotMechSpdFilteredAbs_rads/1
  Zero3/1 -> VfMDAS_SelectedElecAngle_rad/1

== system YMBOX_Control_Core/MDAS/MDAS_DriveModeRoute_Variant/MDAS_Route_SMO/Action_IF_Startup ==
  note: delta_cpr_err
  VfMDAS_SourceMechSpd_rads : Inport
  VfMDAS_SourceMechSpdAbs_rads : Inport  Port=2
  VfMDAS_SourceElecAngle_rad : Inport  Port=3
  Action Port : ActionPort  ActionPortLabel=case [ 16 ]:
  VfMDAS_MotMechSpdFiltered_rads : Outport
  VfMDAS_MotMechSpdFilteredAbs_rads : Outport  Port=2
  VfMDAS_SelectedElecAngle_rad : Outport  Port=3
  wires:
  VfMDAS_SourceMechSpd_rads/1 -> VfMDAS_MotMechSpdFiltered_rads/1
  VfMDAS_SourceMechSpdAbs_rads/1 -> VfMDAS_MotMechSpdFilteredAbs_rads/1
  VfMDAS_SourceElecAngle_rad/1 -> VfMDAS_SelectedElecAngle_rad/1

== system YMBOX_Control_Core/MDAS/MDAS_DriveModeRoute_Variant/MDAS_Route_SMO/Action_SMO_ClosedLoop ==
  note: delta_cpr_err
  VfMDAS_SourceMechSpd_rads : Inport
  VfMDAS_SourceMechSpdAbs_rads : Inport  Port=2
  VfMDAS_SourceElecAngle_rad : Inport  Port=3
  Action Port : ActionPort  ActionPortLabel=case [ 17 ]:
  VfMDAS_MotMechSpdFiltered_rads : Outport
  VfMDAS_MotMechSpdFilteredAbs_rads : Outport  Port=2
  VfMDAS_SelectedElecAngle_rad : Outport  Port=3
  wires:
  VfMDAS_SourceMechSpd_rads/1 -> VfMDAS_MotMechSpdFiltered_rads/1
  VfMDAS_SourceMechSpdAbs_rads/1 -> VfMDAS_MotMechSpdFilteredAbs_rads/1
  VfMDAS_SourceElecAngle_rad/1 -> VfMDAS_SelectedElecAngle_rad/1

== system YMBOX_Control_Core/MDAS/MDAS_DriveModeRoute_Variant/MDAS_Route_SMO/Switch Case Action Subsystem ==
  note: delta_cpr_err
  VuMDSP_MotMechAngleRaw_NULL : Inport
  Action Port : ActionPort  InitializeStates=reset  ActionPortLabel=case [ 1 2 3 4 5 ]:
  Abs1 : Abs  SaturateOnIntegerOverflow=off
  Cast To Double : DataTypeConversion  OutDataTypeStr=single  SaturateOnIntegerOverflow=off  RndMeth=Floor
  Constant1 : Constant  Value=KfPLL_ControlAngleCounts_NULL
  Constant14 : Constant  Value=KfPLL_Bandwidth_rads*KfPLL_Bandwidth_rads
  Constant3 : Constant  Value=KfPLL_PositionCountsPerRev_NULL
  Constant4 : Constant  Value=KfPLL_OneByFreq_s
  Constant5 : Constant  Value=KfPLL_OneByFreq_s
  Constant6 : Constant  Value=KfPLL_OneByFreq_s
  ControlCount_To_ElecAngleRad : Gain  Gain=KfMDAS_ControlCountToElecRad_NULL  OutDataTypeStr=single
  Delay3 : Delay  DelayLength=1  InputProcessing=Columns as channels (frame based)
  Delay4 : Delay  DelayLength=1  InitialConditionSource=Input port  InputProcessing=Columns as channels (frame based)
      settings: InputPortMap=u0,p4
  Divide2 : Product  Inputs=**
  Floor1 : Rounding
  Gain : Gain  Gain=KfPLL_CountToMechRad_radpercnt
  Gain1 : Gain  Gain=2*KfPLL_Bandwidth_rads
  Gain2 : Gain  Gain=KfPLL_PolePairsNativeToControl_NULL
  If2 : If  IfExpression=u1 > KfPLL_HalfPositionCounts_NULL  ElseIfExpressions=u1 < -KfPLL_HalfPositionCounts_NULL
  Merge2 : Merge  Inputs=3
  Minus2 : Sum
  Minus4 : Sum  Inputs=-+
  Minus5 : Sum
  Mod : Math  Operator=mod
  Mod1 : Math  Operator=mod
  Plus1 : Sum
  Product : Product
  Product1 : Product
  Product3 : Product
  Signal Conversion : SignalConversion  OverrideOpt=off
  Switch Case Action Subsystem6 : Subsystem  TreatAsAtomicUnit=on
  Switch Case Action Subsystem7 : Subsystem  TreatAsAtomicUnit=on
  Switch Case Action Subsystem8 : Subsystem  TreatAsAtomicUnit=on
  VfMDAS_MotMechSpdFiltered_rads : Outport
  VfMDAS_MotMechSpdFilteredAbs_rads : Outport  Port=2
  VfMDAS_SelectedElecAngle_rad : Outport  Port=3
  wires:
  If2/2 -> Switch Case Action Subsystem7/Action
  Minus2/1 -> Plus1/1, Floor1/1  "pos_cpr_hat_pred"
  Minus4/1 -> [delta_pre], If2/1
  VuMDSP_MotMechAngleRaw_NULL/1 -> Cast To Double/1
  Merge2/1 -> Product/1, Gain1/1  "delta_cpr_err"
  Divide2/1 -> Minus2/1
  Switch Case Action Subsystem6/1(Out1) -> Merge2/1
  [delta_pre] -> Switch Case Action Subsystem7/1(In1)
  Constant5/1 -> Product3/2
  Delay3/1 -> Divide2/2, Minus5/1  "vel_hat_count"
  Gain1/1 -> Product1/1
  Plus1/1 -> Gain2/1, Mod1/1
  [delta_pre] -> Switch Case Action Subsystem8/1(In1)
  If2/3 -> Switch Case Action Subsystem8/Action
  Cast To Double/1 -> Delay4/2, Minus4/2
  Delay4/1 -> Minus2/2  "pos_cpr_hat_count"
  Product/1 -> Product3/1
  Constant6/1 -> Divide2/1
  Constant14/1 -> Product/2
  If2/1 -> Switch Case Action Subsystem6/Action
  Constant4/1 -> Product1/2
  Switch Case Action Subsystem8/1(Out1) -> Merge2/3
  Product3/1 -> Minus5/2
  Switch Case Action Subsystem7/1(Out1) -> Merge2/2
  [delta_pre] -> Switch Case Action Subsystem6/1(In1)
  Product1/1 -> Plus1/2
  Gain/1 -> Signal Conversion/1, Abs1/1
  Abs1/1 -> VfMDAS_MotMechSpdFilteredAbs_rads/1
  Minus5/1 -> Gain/1, Delay3/1
  Signal Conversion/1 -> VfMDAS_MotMechSpdFiltered_rads/1
  ControlCount_To_ElecAngleRad/1 -> VfMDAS_SelectedElecAngle_rad/1
  Floor1/1 -> Minus4/1
  Gain2/1 -> Mod/1
  Constant1/1 -> Mod/2
  Mod/1 -> ControlCount_To_ElecAngleRad/1
  Constant3/1 -> Mod1/2
  Mod1/1 -> Delay4/1

== system YMBOX_Control_Core/MDAS/MDAS_DriveModeRoute_Variant/MDAS_Route_SensoredOnly/Sensored_AngleSpeed ==
  note: delta_cpr_err
  VuMDSP_MotMechAngleRaw_NULL : Inport
  Reset : ResetPort  DisableCoverage=on
  Abs1 : Abs  SaturateOnIntegerOverflow=off
  Cast To Double : DataTypeConversion  OutDataTypeStr=single  SaturateOnIntegerOverflow=off  RndMeth=Floor
  Constant1 : Constant  Value=KfPLL_ControlAngleCounts_NULL
  Constant14 : Constant  Value=KfPLL_Bandwidth_rads*KfPLL_Bandwidth_rads
  Constant3 : Constant  Value=KfPLL_PositionCountsPerRev_NULL
  Constant4 : Constant  Value=KfPLL_OneByFreq_s
  Constant5 : Constant  Value=KfPLL_OneByFreq_s
  Constant6 : Constant  Value=KfPLL_OneByFreq_s
  ControlCount_To_ElecAngleRad : Gain  Gain=KfMDAS_ControlCountToElecRad_NULL  OutDataTypeStr=single
  Delay3 : Delay  DelayLength=1  InputProcessing=Columns as channels (frame based)
  Delay4 : Delay  DelayLength=1  InitialConditionSource=Input port  InputProcessing=Columns as channels (frame based)
      settings: InputPortMap=u0,p4
  Divide2 : Product  Inputs=**
  Floor1 : Rounding
  Gain : Gain  Gain=KfPLL_CountToMechRad_radpercnt
  Gain1 : Gain  Gain=2*KfPLL_Bandwidth_rads
  Gain2 : Gain  Gain=KfPLL_PolePairsNativeToControl_NULL
  If2 : If  IfExpression=u1 > KfPLL_HalfPositionCounts_NULL  ElseIfExpressions=u1 < -KfPLL_HalfPositionCounts_NULL
  Merge2 : Merge  Inputs=3
  Minus2 : Sum
  Minus4 : Sum  Inputs=-+
  Minus5 : Sum
  Mod : Math  Operator=mod
  Mod1 : Math  Operator=mod
  Plus1 : Sum
  Product : Product
  Product1 : Product
  Product3 : Product
  Signal Conversion : SignalConversion  OverrideOpt=off
  Switch Case Action Subsystem6 : Subsystem  TreatAsAtomicUnit=on
  Switch Case Action Subsystem7 : Subsystem  TreatAsAtomicUnit=on
  Switch Case Action Subsystem8 : Subsystem  TreatAsAtomicUnit=on
  VfMDAS_MotMechSpdFiltered_rads : Outport
  VfMDAS_MotMechSpdFilteredAbs_rads : Outport  Port=2
  VfMDAS_SelectedElecAngle_rad : Outport  Port=3
  wires:
  Signal Conversion/1 -> VfMDAS_MotMechSpdFiltered_rads/1
  Minus5/1 -> Delay3/1, Gain/1
  Abs1/1 -> VfMDAS_MotMechSpdFilteredAbs_rads/1
  Gain/1 -> Abs1/1, Signal Conversion/1
  Product1/1 -> Plus1/2
  [delta_pre] -> Switch Case Action Subsystem6/1(In1)
  Switch Case Action Subsystem7/1(Out1) -> Merge2/2
  Product3/1 -> Minus5/2
  Switch Case Action Subsystem8/1(Out1) -> Merge2/3
  Constant4/1 -> Product1/2
  If2/1 -> Switch Case Action Subsystem6/Action
  Constant14/1 -> Product/2
  Constant6/1 -> Divide2/1
  Product/1 -> Product3/1
  Delay4/1 -> Minus2/2  "pos_cpr_hat_count"
  Cast To Double/1 -> Delay4/2, Minus4/2
  If2/3 -> Switch Case Action Subsystem8/Action
  [delta_pre] -> Switch Case Action Subsystem8/1(In1)
  Plus1/1 -> Gain2/1, Mod1/1
  Gain1/1 -> Product1/1
  Delay3/1 -> Minus5/1, Divide2/2  "vel_hat_count"
  Constant5/1 -> Product3/2
  [delta_pre] -> Switch Case Action Subsystem7/1(In1)
  Switch Case Action Subsystem6/1(Out1) -> Merge2/1
  Divide2/1 -> Minus2/1
  Merge2/1 -> Gain1/1, Product/1  "delta_cpr_err"
  VuMDSP_MotMechAngleRaw_NULL/1 -> Cast To Double/1
  Minus4/1 -> If2/1, [delta_pre]
  Minus2/1 -> Plus1/1, Floor1/1  "pos_cpr_hat_pred"
  If2/2 -> Switch Case Action Subsystem7/Action
  ControlCount_To_ElecAngleRad/1 -> VfMDAS_SelectedElecAngle_rad/1
  Floor1/1 -> Minus4/1
  Gain2/1 -> Mod/1
  Constant1/1 -> Mod/2
  Mod/1 -> ControlCount_To_ElecAngleRad/1
  Constant3/1 -> Mod1/2
  Mod1/1 -> Delay4/1

== system YMBOX_Control_Core/MDAS/Sensorless_FluxMRAS/Observer_Variant1_SMO/Observer_RunState ==
  MDSM_outputs : Inport
  IfMode : Constant  Value=uint16(16)
  InSensorlessFamily : Logic  Operator=OR  IconShape=distinctive
  IsIf : RelationalOperator  Operator===
  IsSmo : RelationalOperator  Operator===
  Mode : BusSelector  OutputSignals=VeMDSM_DrvModeCmd_enum
  SmoMode : Constant  Value=uint16(17)
  Active : Outport
  wires:
  InSensorlessFamily/1 -> Active/1
  SmoMode/1 -> IsSmo/2
  MDSM_outputs/1 -> Mode/1
  Mode/1 -> IsSmo/1, IsIf/1  "<VeMDSM_DrvModeCmd_enum>"
  IfMode/1 -> IsIf/2
  IsIf/1 -> InSensorlessFamily/1
  IsSmo/1 -> InSensorlessFamily/2

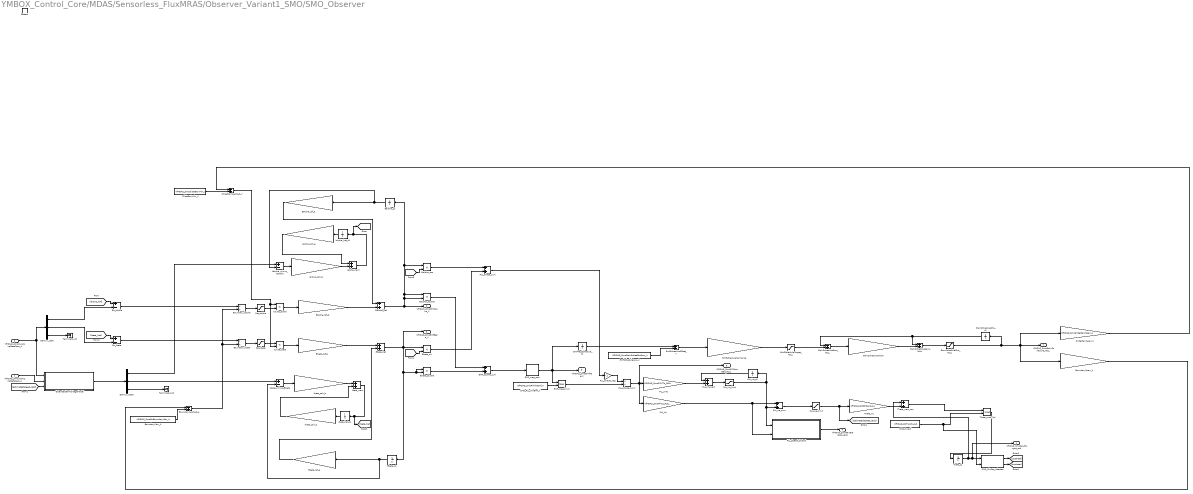
== system YMBOX_Control_Core/MDAS/Sensorless_FluxMRAS/Observer_Variant1_SMO/SMO_Observer ==
  VfMDAS_SmoVoltAlphaBetaZero_V : Inport
  VfMDAS_SmoCurAlphaBetaZero_A : Inport  Port=2  OutDataTypeStr=single
  Restart : ResetPort  DisableCoverage=on
  BoundaryApplied_A : Sum  Inputs=-+
  BoundaryMax_A : Constant  Value=KfMDAS_SmoErrBoundaryMax_A
  BoundarySpan_A : Gain  Gain=KfMDAS_SmoErrBoundarySpan_A
  Boundary_Ialpha : Product  Inputs=*/
  Boundary_Ibeta : Product  Inputs=*/
  Demux_Iab0 : Demux  Outputs=3
  Demux_Uab0 : Demux  Outputs=3
  EMF_mag_limit : MinMax  Function=max  Inputs=2
  EMF_mag_sqrt : YMBOX_SharedMath_Lib/Sqrt_Service  SystemSampleTime=-1  VariantActivationTime=update diagram  AllowFlexibleInterface=on  Latency=0  AutoFrameSizeCalculation=off
  EMF_square_sum : Sum
  Ealpha_cos : Product  Inputs=**
  Ealpha_hat : Sum
  Ealpha_lpf_a : Gain  Gain=KfMDAS_SmoEmfLpfCoefA_NULL
  Ealpha_lpf_b : Gain  Gain=KfMDAS_SmoEmfLpfCoefB_NULL
  Ealpha_square : Product  Inputs=**
  Ealpha_z1 : UnitDelay  InitialCondition=single(0)  SampleTime=-1  HasFrameUpgradeWarning=on
  Ebeta_hat : Sum
  Ebeta_lpf_a : Gain  Gain=KfMDAS_SmoEmfLpfCoefA_NULL
  Ebeta_lpf_b : Gain  Gain=KfMDAS_SmoEmfLpfCoefB_NULL
  Ebeta_sin : Product  Inputs=**
  Ebeta_square : Product  Inputs=**
  Ebeta_z1 : UnitDelay  InitialCondition=single(0)  SampleTime=-1  HasFrameUpgradeWarning=on
  EmfMagSchedule_z1 : UnitDelay  InitialCondition=single(0)  SampleTime=-1
  EmfScheduleLow_V : Constant  Value=KfMDAS_SmoGainSchedEmfLow_V
  EmfScheduleNormalize : Gain  Gain=KfMDAS_SmoGainSchedInvSpan_PerV
  EmfScheduleOffset_V : Sum  Inputs=+-
  EmfScheduleTarget_NULL : Saturate  UpperLimit=1  LowerLimit=0
  Err_Ialpha : Sum  Inputs=+-
  Err_Ibeta : Sum  Inputs=+-
  ExtendedEmfVoltageModel : Subsystem
  GainScheduleAlpha : Gain  Gain=KfMDAS_SmoGainSchedAlpha_NULL
  GainScheduleError_NULL : Sum  Inputs=-+
  GainScheduleNext_NULL : Sum
  GainScheduleRho_NULL : Saturate  UpperLimit=1  LowerLimit=0
  GainScheduleRho_z1 : UnitDelay  InitialCondition=single(0)  SampleTime=-1
  Ialpha_hat_z1 : UnitDelay  InitialCondition=single(0)  SampleTime=-1  HasFrameUpgradeWarning=on
  Ialpha_next : Sum
  Ialpha_zoh_a : Gain  Gain=KfMDAS_SmoCurrentZohCoefA_NULL
  Ialpha_zoh_b : Gain  Gain=KfMDAS_SmoCurrentZohCoefB_AperV
  Ibeta_hat_z1 : UnitDelay  InitialCondition=single(0)  SampleTime=-1  HasFrameUpgradeWarning=on
  Ibeta_next : Sum
  Ibeta_zoh_a : Gain  Gain=KfMDAS_SmoCurrentZohCoefA_NULL
  Ibeta_zoh_b : Gain  Gain=KfMDAS_SmoCurrentZohCoefB_AperV
  Kslide_alpha : Product  Inputs=**
  Kslide_beta : Product  Inputs=**
  PLL_KiTs : Gain  Gain=KfMDAS_SmoPllKiTs_NULL
  PLL_Kp : Gain  Gain=KfMDAS_SmoPllKp_NULL
  PLL_Speed_Output : Subsystem  Description=Speed estimate = PLL integral state + low-pass proportional correction. Filter pole Ki/Kp, alpha = 1-exp(-KiTs/Kp). Constant acceleration correction is retained while fast proportional ripple is attenuated.
  PLL_int_limit : Saturate  UpperLimit=KfMDAS_SlsElecSpdMax_rads  LowerLimit=KfMDAS_SlsElecSpdMin_rads
  PLL_int_next : Sum
  PLL_int_z1 : UnitDelay  InitialCondition=single(0)  SampleTime=-1  HasFrameUpgradeWarning=on
  PLL_phase_neg : Gain  Gain=-1
  PLL_phase_norm : Product  Inputs=*/
  PLL_phase_sum : Sum
  PLL_we_limit : Saturate  UpperLimit=KfMDAS_SlsElecSpdMax_rads  LowerLimit=KfMDAS_SlsElecSpdMin_rads
  PLL_we_sum : Sum
  SMO_PLL_MinEmf_V : Constant  Value=KfMDAS_SmoPllMinEmf_V  OutDataTypeStr=single
  SMO_SinCos_Adapter : Subsystem
  SMO_TwoPi : Constant  Value=KfMDAS_SlsTwoPi_rad  OutDataTypeStr=single
  Sat_Ialpha : Saturate  UpperLimit=1  LowerLimit=-1
  Sat_Ibeta : Saturate  UpperLimit=1  LowerLimit=-1
  SlideGainApplied_V : Sum
  SlideGainMin_V : Constant  Value=KfMDAS_SmoSlideGainMin_V
  SlideGainSpan_V : Gain  Gain=KfMDAS_SmoSlideGainSpan_V
  Terminator_I0 : Terminator
  Terminator_U0 : Terminator
  Theta_Ts : Gain  Gain=KfMDAS_SlsCtrlPeriod_s
  Theta_mod_2pi : Math  Operator=mod
  Theta_next_raw : Sum
  Ualpha_minus_Ealpha : Sum  Inputs=+-
  Ubeta_minus_Ebeta : Sum  Inputs=+-
  theta_z1 : UnitDelay  InitialCondition=single(KfMDAS_SlsEAngleInit_rad)  SampleTime=-1  HasFrameUpgradeWarning=on
  VfMDAS_SmoRawEAngle_rad : Outport  OutDataTypeStr=single
  VfMDAS_SmoEmfAlpha_V : Outport  Port=2  OutDataTypeStr=single
  VfMDAS_SmoEmfBeta_V : Outport  Port=3  OutDataTypeStr=single
  VfMDAS_SmoRawElecSpd_rads : Outport  Description=Publish the PLL integral speed plus the filtered proportional acceleration correction. Internal angle propagation retains the unfiltered proportional-plus-integral speed.  Port=4  OutDataTypeStr=single
  VfMDAS_SmoEmfMag_V : Outport  Port=5
  VfMDAS_SmoPllPhaseErr_NULL : Outport  Port=6
  VfMDAS_SmoGainSchedule_NULL : Outport  Port=7
  wires:
  PLL_phase_sum/1 -> PLL_phase_neg/1
  SlideGainSpan_V/1 -> SlideGainApplied_V/1
  Ebeta_z1/1 -> Ebeta_lpf_a/1, Ubeta_minus_Ebeta/2
  PLL_phase_norm/1 -> PLL_KiTs/1, PLL_Kp/1, VfMDAS_SmoPllPhaseErr_NULL/1
  PLL_phase_neg/1 -> PLL_phase_norm/1
  Demux_Iab0/2 -> Err_Ibeta/2
  PLL_KiTs/1 -> PLL_int_next/2
  Demux_Iab0/1 -> Err_Ialpha/2
  Ebeta_sin/1 -> PLL_phase_sum/2
  PLL_int_z1/1 -> PLL_int_next/1
  PLL_int_next/1 -> PLL_int_limit/1
  PLL_Kp/1 -> PLL_we_sum/1, PLL_Speed_Output/2(ProportionalCorrection_rads)
  PLL_int_limit/1 -> PLL_int_z1/1, PLL_Speed_Output/1(IntegralSpeed_rads), PLL_we_sum/2
  SlideGainMin_V/1 -> SlideGainApplied_V/2
  Err_Ialpha/1 -> Boundary_Ialpha/1
  PLL_Speed_Output/1(Speed_rads) -> VfMDAS_SmoRawElecSpd_rads/1
  Demux_Uab0/2 -> Ubeta_minus_Ebeta/1
  Demux_Uab0/1 -> Ualpha_minus_Ealpha/1
  Theta_Ts/1 -> Theta_next_raw/2
  PLL_we_sum/1 -> PLL_we_limit/1
  Ealpha_z1/1 -> Ualpha_minus_Ealpha/2, Ealpha_lpf_a/1
  Ualpha_minus_Ealpha/1 -> Ialpha_zoh_b/1
  Kslide_beta/1 -> Ebeta_lpf_b/1
  Ubeta_minus_Ebeta/1 -> Ibeta_zoh_b/1
  Ealpha_square/1 -> EMF_square_sum/1
  SlideGainApplied_V/1 -> Kslide_alpha/1, Kslide_beta/2  "VfMDAS_SmoSlideGainApplied_V"
  Sat_Ialpha/1 -> Kslide_alpha/2
  Sat_Ibeta/1 -> Kslide_beta/1
  Ealpha_cos/1 -> PLL_phase_sum/1
  EMF_mag_limit/1 -> PLL_phase_norm/2
  Ialpha_zoh_a/1 -> Ialpha_next/1
  PLL_we_limit/1 -> Theta_Ts/1, [estimatedSpeed_rads]
  Kslide_alpha/1 -> Ealpha_lpf_b/1
  Ealpha_hat/1 -> Ealpha_z1/1, Ealpha_cos/1, Ealpha_square/1, Ealpha_square/2, VfMDAS_SmoEmfAlpha_V/1
  VfMDAS_SmoVoltAlphaBetaZero_V/1 -> ExtendedEmfVoltageModel/2(appliedVoltageAb0_V)
  theta_z1/1 -> VfMDAS_SmoRawEAngle_rad/1, SMO_SinCos_Adapter/1(thetaRad), Theta_next_raw/1
  EmfScheduleLow_V/1 -> EmfScheduleOffset_V/2
  Ialpha_zoh_b/1 -> Ialpha_next/2
  VfMDAS_SmoCurAlphaBetaZero_A/1 -> ExtendedEmfVoltageModel/1(currentAb0_A), Demux_Iab0/1
  Ibeta_zoh_b/1 -> Ibeta_next/1
  BoundaryApplied_A/1 -> Boundary_Ibeta/2, Boundary_Ialpha/2  "VfMDAS_SmoErrBoundaryApplied_A"
  Ibeta_zoh_a/1 -> Ibeta_next/2
  Ealpha_lpf_a/1 -> Ealpha_hat/1
  Ealpha_lpf_b/1 -> Ealpha_hat/2
  SMO_TwoPi/1 -> SMO_SinCos_Adapter/2(twoPiRad), Theta_mod_2pi/2
  ExtendedEmfVoltageModel/1(equivalentVoltageAb0_V) -> Demux_Uab0/1
  Demux_Iab0/3 -> Terminator_I0/1
  Ialpha_next/1 -> Ialpha_hat_z1/1, [Ialpha_hat]
  Ibeta_next/1 -> Ibeta_hat_z1/1, [Ibeta_hat]
  Ebeta_hat/1 -> VfMDAS_SmoEmfBeta_V/1, Ebeta_sin/1, Ebeta_z1/1, Ebeta_square/2, Ebeta_square/1
  Ebeta_lpf_a/1 -> Ebeta_hat/2
  Ebeta_lpf_b/1 -> Ebeta_hat/1
  Ialpha_hat_z1/1 -> Ialpha_zoh_a/1
  Demux_Uab0/3 -> Terminator_U0/1
  Ebeta_square/1 -> EMF_square_sum/2
  Ibeta_hat_z1/1 -> Ibeta_zoh_a/1
  SMO_PLL_MinEmf_V/1 -> EMF_mag_limit/2
  Err_Ibeta/1 -> Boundary_Ibeta/1
  EmfMagSchedule_z1/1 -> EmfScheduleOffset_V/1
  EmfScheduleOffset_V/1 -> EmfScheduleNormalize/1
  EmfScheduleNormalize/1 -> EmfScheduleTarget_NULL/1
  GainScheduleRho_z1/1 -> GainScheduleError_NULL/1, GainScheduleNext_NULL/1
  EmfScheduleTarget_NULL/1 -> GainScheduleError_NULL/2
  GainScheduleError_NULL/1 -> GainScheduleAlpha/1
  GainScheduleAlpha/1 -> GainScheduleNext_NULL/2
  GainScheduleNext_NULL/1 -> GainScheduleRho_NULL/1
  GainScheduleRho_NULL/1 -> VfMDAS_SmoGainSchedule_NULL/1, SlideGainSpan_V/1, BoundarySpan_A/1, GainScheduleRho_z1/1  "VfMDAS_SmoGainSchedule_NULL"
  BoundarySpan_A/1 -> BoundaryApplied_A/1
  BoundaryMax_A/1 -> BoundaryApplied_A/2
  Boundary_Ialpha/1 -> Sat_Ialpha/1
  Boundary_Ibeta/1 -> Sat_Ibeta/1
  [Ialpha_hat] -> Err_Ialpha/1
  [estimatedSpeed_rads] -> ExtendedEmfVoltageModel/3(estimatedSpeed_rads)
  [Ibeta_hat] -> Err_Ibeta/1
  SMO_SinCos_Adapter/1(cosTheta) -> [costheta]
  [costheta] -> Ealpha_cos/2
  SMO_SinCos_Adapter/2(sinTheta) -> [sintheta]
  [sintheta] -> Ebeta_sin/2
  EMF_square_sum/1 -> EMF_mag_sqrt/1
  EMF_mag_sqrt/1 -> EmfMagSchedule_z1/1, EMF_mag_limit/1, VfMDAS_SmoEmfMag_V/1  "VfMDAS_SmoEmfMagSchedule_V"
  Theta_next_raw/1 -> Theta_mod_2pi/1
  Theta_mod_2pi/1 -> theta_z1/1

== system YMBOX_Control_Core/MDAS/Sensorless_FluxMRAS/Observer_Variant1_SMO/SMO_RotationDirectionOffset ==
  electricalSpeed : Inport
  Pi : Constant  Value=single(0.5*KfMDAS_SlsTwoPi_rad)  OutDataTypeStr=single
  Select : Switch
  Zero : Constant  Value=single(0)  OutDataTypeStr=single
  angleOffset : Outport
  wires:
  Zero/1 -> Select/1
  electricalSpeed/1 -> Select/2
  Pi/1 -> Select/3
  Select/1 -> angleOffset/1
